simulink library "Pitch_Controller_Lib"  (R2025a)
settings: Solver=ode45  StartTime=0.0  StopTime=10.0  RelTol=1e-3  EnableMultiTasking=on
undefined symbols (not defined in the file or in its folder): Actuator_Lookup, P_VAR_Blade_Length, P_VAR_emergency_brake_pitch_angle, P_VAR_LUT_max_pitch_angle, P_VAR_park_pitch_angle, P_VAR_Rotor_nominal_rpm, PARAM_PCTRL_alpha_Igain, PARAM_PCTRL_alpha_Pgain, PARAM_PCTRL_Dgain, PARAM_PCTRL_Igain, PARAM_PCTRL_Pgain, radps2rpm, WT_Params
libraries: $bdroot x1
Description:
  | Copyright 2009-2025 The MathWorks, Inc.
settings Model: Creator=smiller  LastModifiedBy=smiller
settings SolverCC: AlgebraicLoopSolver=TrustRegion
settings DataIOCC: LimitDataPoints=on  SaveFormat=Array  SignalLoggingSaveFormat=ModelDataLogs  ReturnWorkspaceOutputs=off
settings OptimizationCC: ReuseModelBlockBuffer=off  ExpressionDepthLimit=2147483647.0  LifeSpan=inf
settings DebuggingCC: UnderspecifiedInitializationDetection=Classic  MergeDetectMultiDrivingBlocksExec=none  SolverPrmCheckMsg=warning  FcnCallInpInsideContextMsg=warning  UnconnectedInputMsg=warning  UnconnectedOutputMsg=warning  UnconnectedLineMsg=warning  AllowSymbolicDim=off  StateNameClashWarn=warning  PregeneratedLibrarySubsystemCodeDiagnostic=none  SFUnexpectedBacktrackingDiag=warning  SFNoUnconditionalDefaultTransitionDiag=warning  SFExecutionAtInitializationDiag=none  ArithmeticOperatorsInVariantConditions=warning
settings HardwareCC: ProdBitPerPointer=32.0  ProdBitPerSizeT=32.0  ProdBitPerPtrDiffT=32.0  ProdLargestAtomicFloat=None  ProdIntDivRoundTo=Undefined  ProdEndianess=Unspecified  ProdWordSize=32.0  ProdHWDeviceType=32-bit Generic
settings ModelReferenceCC: EnableRefExpFcnMdlSchedulingChecks=on  PropagateSignalLabelsOutOfModel=off
settings SFSimCC: SimUseLocalCustomCode=off  CustomCodeUndefinedFunction=UseInterfaceOnly
settings RTWCC: RTWUseLocalCustomCode=off  GPUComputeCapability=3.5  DLArmComputeVersion=19.05
settings CodeAppCC: StateflowObjectComments=on
settings GRTTargetCC: TargetLangStandard=C89/C90 (ANSI)  CombineOutputUpdateFcns=off  GRTInterface=on
settings ConfigComp: CovMetricSettings=dw  CovSaveCumulativeToWorkspaceVar=on  CovSaveSingleToWorkspaceVar=on  CovExternalEMLEnable=off  CovSFcnEnable=off

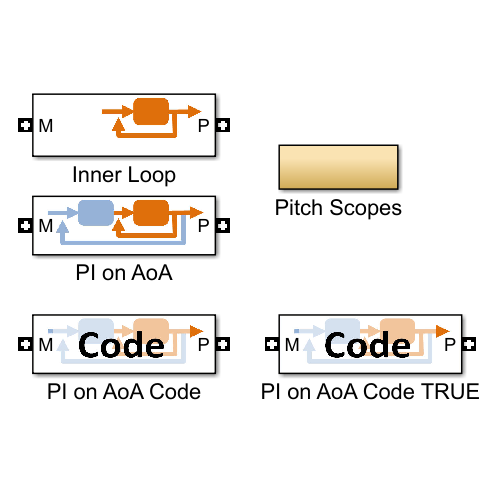
[thumbnail: Simulink's stored preview of the top-level diagram]
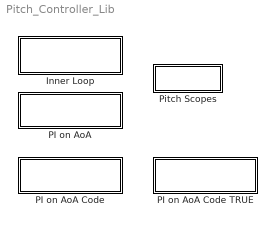
== system Pitch_Controller_Lib ==
  Inner Loop : Subsystem
      mask Display: image('Pitch_Controller_Inner_Loop_IMAGE.jpg');
  PI on AoA : Subsystem
      mask Display: image('Pitch_Controller_PI_on_AOA_IMAGE.jpg');
  PI on AoA Code : Subsystem
      mask Display: image('Pitch_Controller_PI_on_AOA_S_Function_IMAGE.jpg');
  PI on AoA Code TRUE : Subsystem
      mask Display: image('Pitch_Controller_PI_on_AOA_S_Function_IMAGE.jpg');
  Pitch Scopes : Subsystem

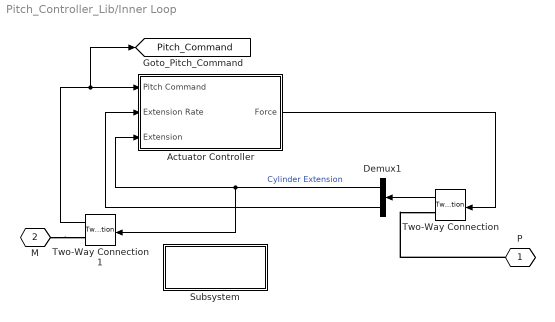
== system Pitch_Controller_Lib/Inner Loop ==
  Actuator Controller : Subsystem
  Demux1 : Demux  Outputs=2
  Subsystem : Subsystem
      mask Display: disp('Inner loop')
  Two-Way Connection : TwoWayConnection
  Two-Way Connection1 : TwoWayConnection
  P : PMIOPort  Tag=PMCPort  Side=Right
  M : PMIOPort  Tag=PMCPort  Port=2  Side=Left
  tag scope: Pitch_Command=global
  wires:
  Actuator Controller/1(Force) -> Two-Way Connection/1
  Demux1/2 -> Actuator Controller/2(Extension Rate)
  Demux1/1 -> Two-Way Connection1/1, Actuator Controller/3(Extension)  "Cylinder Extension"
  Two-Way Connection/1 -> Demux1/1
  Two-Way Connection1/1 -> [Pitch_Command], Actuator Controller/1(Pitch Command)
  connections:
  M/RConn1 -- Two-Way Connection1/RConn1
  P/RConn1 -- Two-Way Connection/RConn1

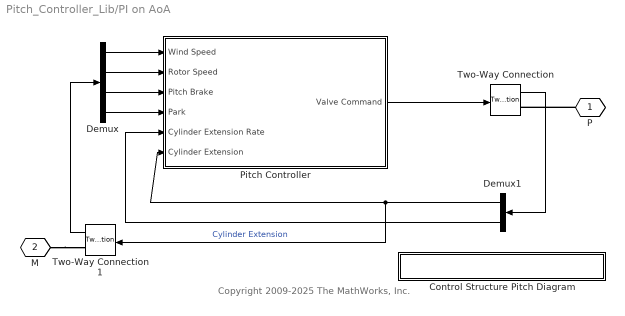
== system Pitch_Controller_Lib/PI on AoA ==
  note: Copyright 2009-2025 The MathWorks, Inc.
  Control Structure Pitch Diagram : Subsystem
      mask Display: disp('View Pitch Control Structure');
  Demux : Demux
  Demux1 : Demux  Outputs=2
  Pitch Controller : Subsystem
  Two-Way Connection : TwoWayConnection
  Two-Way Connection1 : TwoWayConnection
  P : PMIOPort  Tag=PMCPort  Side=Right
  M : PMIOPort  Tag=PMCPort  Port=2  Side=Left
  wires:
  Pitch Controller/1(Valve Command) -> Two-Way Connection/1
  Two-Way Connection/1 -> Demux1/1
  Demux1/2 -> Pitch Controller/5(Cylinder Extension Rate)
  Demux1/1 -> Two-Way Connection1/1, Pitch Controller/6(Cylinder Extension)  "Cylinder Extension"
  Two-Way Connection1/1 -> Demux/1
  Demux/1 -> Pitch Controller/1(Wind Speed)
  Demux/2 -> Pitch Controller/2(Rotor Speed)
  Demux/3 -> Pitch Controller/3(Pitch Brake)
  Demux/4 -> Pitch Controller/4(Park)
  connections:
  P/RConn1 -- Two-Way Connection/RConn1
  M/RConn1 -- Two-Way Connection1/RConn1

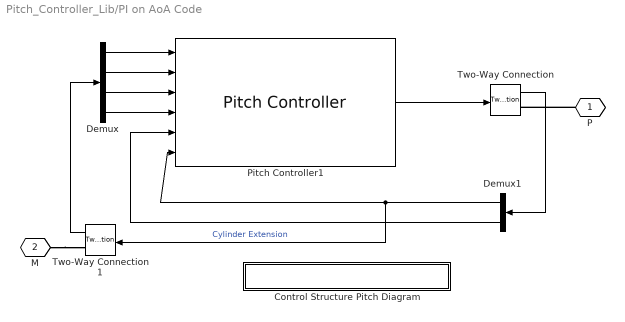
== system Pitch_Controller_Lib/PI on AoA Code ==
  Control Structure Pitch Diagram : Subsystem
      mask Display: disp('View Pitch Control Structure');
  Demux : Demux
  Demux1 : Demux  Outputs=2
  Pitch Controller1 : $bdroot/PI on AoA/Pitch Controller  SystemSampleTime=-1  VariantActivationTime=update diagram  EmptyChoice=off  PassThrough=off  PassThroughVariantControl=(default)  EmptyChoiceVariantControl=(default)  AllowFlexibleInterface=on  Latency=0  AutoFrameSizeCalculation=off
  Two-Way Connection : TwoWayConnection
  Two-Way Connection1 : TwoWayConnection
  P : PMIOPort  Tag=PMCPort  Side=Right
  M : PMIOPort  Tag=PMCPort  Port=2  Side=Left
  wires:
  Demux/4 -> Pitch Controller1/4
  Demux/3 -> Pitch Controller1/3
  Demux/2 -> Pitch Controller1/2
  Demux/1 -> Pitch Controller1/1
  Two-Way Connection1/1 -> Demux/1
  Demux1/1 -> Pitch Controller1/6, Two-Way Connection1/1  "Cylinder Extension"
  Demux1/2 -> Pitch Controller1/5
  Two-Way Connection/1 -> Demux1/1
  Pitch Controller1/1 -> Two-Way Connection/1
  connections:
  M/RConn1 -- Two-Way Connection1/RConn1
  P/RConn1 -- Two-Way Connection/RConn1

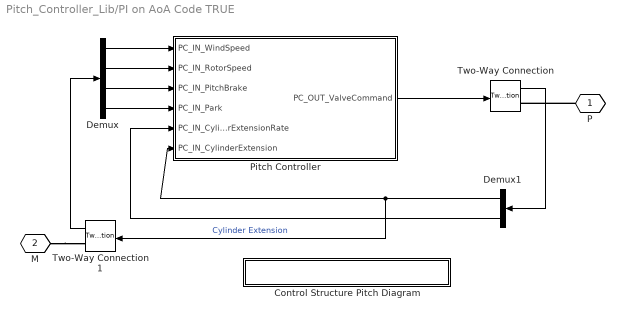
== system Pitch_Controller_Lib/PI on AoA Code TRUE ==
  Control Structure Pitch Diagram : Subsystem
      mask Display: disp('View Pitch Control Structure');
  Demux : Demux
  Demux1 : Demux  Outputs=2
  Pitch Controller : Subsystem
  Two-Way Connection : TwoWayConnection
  Two-Way Connection1 : TwoWayConnection
  P : PMIOPort  Tag=PMCPort  Side=Right
  M : PMIOPort  Tag=PMCPort  Port=2  Side=Left
  wires:
  Pitch Controller/1(PC_OUT_ValveCommand) -> Two-Way Connection/1
  Two-Way Connection/1 -> Demux1/1
  Demux1/2 -> Pitch Controller/5(PC_IN_CylinderExtensionRate)
  Demux1/1 -> Pitch Controller/6(PC_IN_CylinderExtension), Two-Way Connection1/1  "Cylinder Extension"
  Two-Way Connection1/1 -> Demux/1
  Demux/1 -> Pitch Controller/1(PC_IN_WindSpeed)
  Demux/2 -> Pitch Controller/2(PC_IN_RotorSpeed)
  Demux/3 -> Pitch Controller/3(PC_IN_PitchBrake)
  Demux/4 -> Pitch Controller/4(PC_IN_Park)
  connections:
  P/RConn1 -- Two-Way Connection/RConn1
  M/RConn1 -- Two-Way Connection1/RConn1

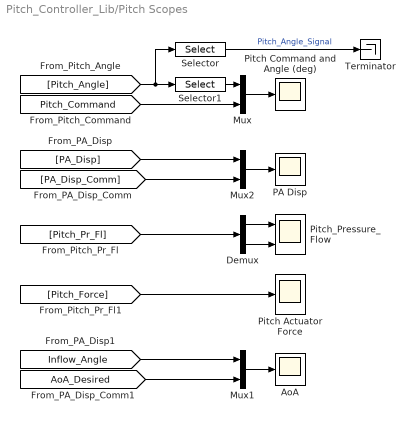
== system Pitch_Controller_Lib/Pitch Scopes ==
  AoA : Scope
      settings: TimeSpan=10  ActiveDisplayYMinimum=-1.6  ActiveDisplayYMaximum=-0.9  DataLoggingVariableName=ScopeData2
  Demux : Demux  Outputs=[2 1]
  Mux : Mux  Inputs=2
  Mux1 : Mux  Inputs=2
  Mux2 : Mux  Inputs=2
  PA Disp : Scope
      settings: TimeSpan=10  ActiveDisplayYMinimum=-1.6  ActiveDisplayYMaximum=-0.9
  Pitch Actuator Force : Scope
      settings: TimeSpan=80  ActiveDisplayYMinimum=-78125  ActiveDisplayYMaximum=84375  DataLoggingVariableName=Pitch_Actuator_Force_DATA
  Pitch Command and Angle (deg) : Scope
      settings: TimeSpan=80  ActiveDisplayYMinimum=-20  ActiveDisplayYMaximum=80  DataLoggingVariableName=Blade_Pitch_DATA
  Pitch_Pressure_Flow : Scope  NumInputPorts=2
      settings: ActiveDisplayYMinimum=-5  ActiveDisplayYMaximum=20  DataLoggingVariableName=ScopeData3
  Selector : Selector  InputPortWidth=3  IndexOptions=Index vector (dialog)  Indices=[1 ]  OutputSizes=1
  Selector1 : Selector  InputPortWidth=3  IndexOptions=Index vector (dialog)  Indices=[1 ]  OutputSizes=1
  Terminator : Terminator
  wires:
  Selector1/1 -> Mux/1
  [Inflow_Angle] -> Mux1/1
  Mux1/1 -> AoA/1
  [AoA_Desired] -> Mux1/2
  [Pitch_Angle] -> Selector1/1, Selector/1
  [Pitch_Command] -> Mux/2
  Mux/1 -> Pitch Command and Angle (deg)/1
  [PA_Disp] -> Mux2/1
  Mux2/1 -> PA Disp/1
  [PA_Disp_Comm] -> Mux2/2
  [Pitch_Pr_Fl] -> Demux/1
  Demux/1 -> Pitch_Pressure_Flow/1
  Demux/2 -> Pitch_Pressure_Flow/2
  Selector/1 -> Terminator/1  "Pitch_Angle_Signal"
  [Pitch_Force] -> Pitch Actuator Force/1

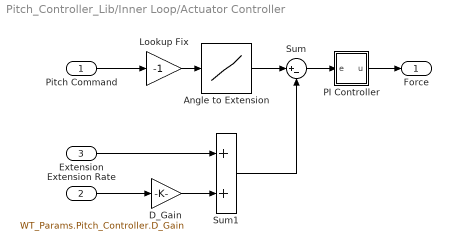
== system Pitch_Controller_Lib/Inner Loop/Actuator Controller ==
  Pitch Command : Inport
  Extension Rate : Inport  Port=2
  Extension : Inport  Port=3
  Angle to Extension : Lookup  InputValues=-Actuator_Lookup.angle  Table=Actuator_Lookup.extension  SaturateOnIntegerOverflow=off
  D_Gain : Gain  Gain=WT_Params.Pitch_Controller.D_Gain
  Lookup Fix : Gain  Gain=-1
  PI Controller : Subsystem
      mask Display: disp('PI')
  Sum : Sum  Inputs=|+-
  Sum1 : Sum
  Force : Outport  VectorParamsAs1DForOutWhenUnconnected=off
  wires:
  Extension Rate/1 -> D_Gain/1
  PI Controller/1(u) -> Force/1
  Extension/1 -> Sum1/1
  Pitch Command/1 -> Lookup Fix/1
  Sum1/1 -> Sum/2
  D_Gain/1 -> Sum1/2
  Lookup Fix/1 -> Angle to Extension/1
  Angle to Extension/1 -> Sum/1
  Sum/1 -> PI Controller/1(e)

== system Pitch_Controller_Lib/Inner Loop/Subsystem ==

== system Pitch_Controller_Lib/PI on AoA/Control Structure Pitch Diagram ==
  Subsystem : Subsystem
      mask Display: image(imread('Control_Structure_Pitch_IMAGE.jpg'));

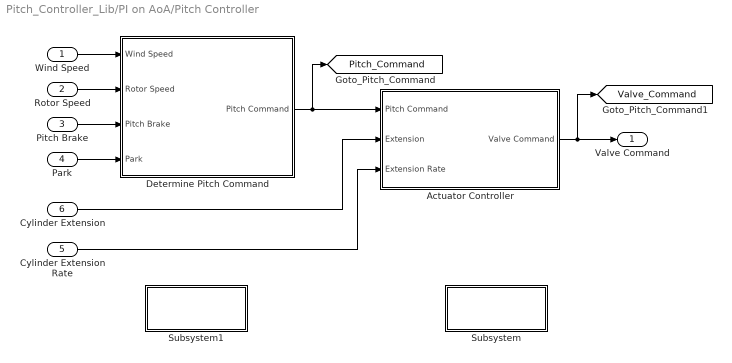
== system Pitch_Controller_Lib/PI on AoA/Pitch Controller ==
  Wind Speed : Inport
  Rotor Speed : Inport  Port=2
  Pitch Brake : Inport  Port=3
  Park : Inport  Port=4
  Cylinder Extension Rate : Inport  Port=5
  Cylinder Extension : Inport  Port=6
  Actuator Controller : Subsystem
  Determine Pitch Command : Subsystem
  Subsystem : Subsystem
      mask Display: disp('Inner loop')
  Subsystem1 : Subsystem
      mask Display: disp('Outer loop')
  Valve Command : Outport  VectorParamsAs1DForOutWhenUnconnected=off
  tag scope: Pitch_Command=global, Valve_Command=global
  wires:
  Determine Pitch Command/1(Pitch Command) -> [Pitch_Command], Actuator Controller/1(Pitch Command)
  Cylinder Extension/1 -> Actuator Controller/2(Extension)
  Wind Speed/1 -> Determine Pitch Command/1(Wind Speed)
  Rotor Speed/1 -> Determine Pitch Command/2(Rotor Speed)
  Actuator Controller/1(Valve Command) -> Valve Command/1, [Valve_Command]
  Pitch Brake/1 -> Determine Pitch Command/3(Pitch Brake)
  Park/1 -> Determine Pitch Command/4(Park)
  Cylinder Extension Rate/1 -> Actuator Controller/3(Extension Rate)

== system Pitch_Controller_Lib/PI on AoA Code/Control Structure Pitch Diagram ==
  Subsystem : Subsystem
      mask Display: image(imread('Control_Structure_Pitch_IMAGE.jpg'));

== system Pitch_Controller_Lib/PI on AoA Code TRUE/Control Structure Pitch Diagram ==
  Subsystem : Subsystem
      mask Display: image(imread('Control_Structure_Pitch_IMAGE.jpg'));

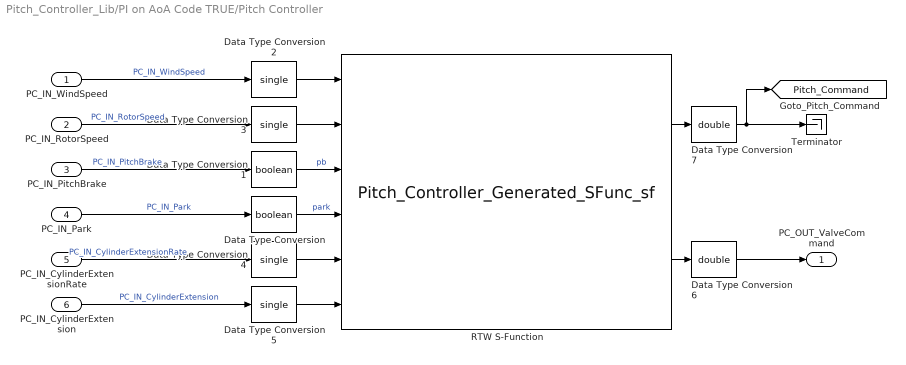
== system Pitch_Controller_Lib/PI on AoA Code TRUE/Pitch Controller ==
  PC_IN_WindSpeed : Inport  OutDataTypeStr=double
  PC_IN_RotorSpeed : Inport  Port=2  OutDataTypeStr=double
  PC_IN_PitchBrake : Inport  Port=3  OutDataTypeStr=double
  PC_IN_Park : Inport  Port=4  OutDataTypeStr=double
  PC_IN_CylinderExtensionRate : Inport  Port=5  OutDataTypeStr=double  PortDimensions=3
  PC_IN_CylinderExtension : Inport  Port=6  OutDataTypeStr=double  PortDimensions=3
  Data Type Conversion : DataTypeConversion  OutDataTypeStr=boolean  SaturateOnIntegerOverflow=off  RndMeth=Floor
  Data Type Conversion1 : DataTypeConversion  OutDataTypeStr=boolean  SaturateOnIntegerOverflow=off  RndMeth=Floor
  Data Type Conversion{2..5} (4 alike) : DataTypeConversion  OutDataTypeStr=single  SaturateOnIntegerOverflow=off  RndMeth=Floor
  Data Type Conversion6 : DataTypeConversion  OutDataTypeStr=double  SaturateOnIntegerOverflow=off  RndMeth=Floor
  Data Type Conversion7 : DataTypeConversion  OutDataTypeStr=double  SaturateOnIntegerOverflow=off  RndMeth=Floor
  RTW S-Function : S-Function  FunctionName=Pitch_Controller_Generated_SFunc_sf  Parameters=sfcnParam1, sfcnParam2, sfcnParam3, sfcnParam4, sfcnParam5, sfcnParam6, sfcnParam7, sfcnParam8, sfcnParam9, sfcnParam10  SFunctionModules=""  SFunctionDeploymentMode=off  EnableBusSupport=off  mask{rtw_sf_name=Pitch_Controller_Generated_SFunc_sf, showVar=off, sfcnParam1=PARAM_PCTRL_Dgain, sfcnParam2=PARAM_PCTRL_Igain, sfcnParam3=PARAM_PCTRL_Pgain, sfcnParam4=PARAM_PCTRL_alpha_Igain, sfcnParam5=PARAM_PCTRL_alpha_Pgain, sfcnParam6=P_VAR_Blade_Length, sfcnParam7=P_VAR_LUT_max_pitch_angle, sfcnParam8=P_VAR_Rotor_nominal_rpm, sfcnParam9=P_VAR_emergency_brake_pitch_angle, sfcnParam10=P_VAR_park_pitch_angle}
      mask prompts: rtw_sf_name "Generated S-function name (model_sf):"; showVar "Show module list"; sfcnParam1 "PARAM_PCTRL_Dgain:"; sfcnParam2 "PARAM_PCTRL_Igain:"; sfcnParam3 "PARAM_PCTRL_Pgain:"; sfcnParam4 "PARAM_PCTRL_alpha_Igain:"; sfcnParam5 "PARAM_PCTRL_alpha_Pgain:"; sfcnParam6 "P_VAR_Blade_Length:"; sfcnParam7 "P_VAR_LUT_max_pitch_angle:"; sfcnParam8 "P_VAR_Rotor_nominal_rpm:"; sfcnParam9 "P_VAR_emergency_brake_pitch_angle:"; sfcnParam10 "P_VAR_park_pitch_angle:"
      mask help: Real-Time Workshop generated S-function.
      mask init:
      | displist = '';
      | if ~strcmp(get_param(gcb, 'FunctionName'), rtw_sf_name);
      |   set_param(gcb, 'FunctionName', rtw_sf_name);
      | end
      | % Check if we are generating RTW code
      | rtw_mode = false;
      | if strcmpi(get_param(bdroot(gcb),'SimulationStatus'),'Initializing')
      | 	rtw_mode = strcmpi(get_param(bdroot(gcb),'BuildingRTWCode'),'on') && ...
      | 		~strcmpi(get_param(bdroot(gcb),'TargetStyle'),'SimulationTarget');
      | end
      | if showVar || rtw_mode
      | 	if exist('rtwsfunc') == 2 | exist('rtwsfunc') == 6
      | 		tmplist = rtwsfunc(rtw_sf_name,gcb);
      | 		tmplist = ['\nList of Modules:\n', tmplist];
      | 	elseif showVar
      | 		tmplist = '\nList of Modules:\nRTW not licensed\n';
      |  	end
      | end
      | if showVar
      |   displist = tmplist;
      | end
      settings: CopyFcn=|
      | if ~strcmp(get_param(gcb,'Linkstatus'),'none') && ...
      | ~strcmp(get_param(gcb,'Linkstatus'),'implicit')
      |   set_param(gcb,'LinkStatus','none');
      | end
      mask Help: eval('feval(''rtwprivate'',''rtwhelpview'',''rtw_sfcn_block'')');
      mask Display:
      | port_label('input',1,'PC_IN_WindSpeed');
      | port_label('input',2,'PC_IN_RotorSpeed');
      | port_label('input',3,'PC_IN_PitchBrake');
      | port_label('input',4,'PC_IN_Park');
      | port_label('input',5,'PC_IN_CylinderExtensionRate');
      | port_label('input',6,'PC_IN_CylinderExtension');
      | port_label('output',1,'PC_LOG_PitchCommand');
      | port_label('output',2,'PC_OUT_ValveCommand');
  Terminator : Terminator
  PC_OUT_ValveCommand : Outport  OutDataTypeStr=double  VectorParamsAs1DForOutWhenUnconnected=off
  tag scope: Pitch_Command=global
  wires:
  Data Type Conversion7/1 -> [Pitch_Command], Terminator/1
  RTW S-Function/1 -> Data Type Conversion7/1
  RTW S-Function/2 -> Data Type Conversion6/1
  Data Type Conversion6/1 -> PC_OUT_ValveCommand/1
  Data Type Conversion5/1 -> RTW S-Function/6
  Data Type Conversion4/1 -> RTW S-Function/5
  Data Type Conversion3/1 -> RTW S-Function/2
  Data Type Conversion2/1 -> RTW S-Function/1
  Data Type Conversion1/1 -> RTW S-Function/3  "pb"
  Data Type Conversion/1 -> RTW S-Function/4  "park"
  PC_IN_CylinderExtension/1 -> Data Type Conversion5/1  "PC_IN_CylinderExtension"
  PC_IN_CylinderExtensionRate/1 -> Data Type Conversion4/1  "PC_IN_CylinderExtensionRate"
  PC_IN_Park/1 -> Data Type Conversion/1  "PC_IN_Park"
  PC_IN_PitchBrake/1 -> Data Type Conversion1/1  "PC_IN_PitchBrake"
  PC_IN_RotorSpeed/1 -> Data Type Conversion3/1  "PC_IN_RotorSpeed"
  PC_IN_WindSpeed/1 -> Data Type Conversion2/1  "PC_IN_WindSpeed"

== system Pitch_Controller_Lib/Inner Loop/Actuator Controller/PI Controller ==
  e : Inport
  Integral Gain : Gain  Gain=WT_Params.Pitch_Controller.I_Gain  SaturateOnIntegerOverflow=on  OutDataTypeStr=Inherit: Same as input  ParamDataTypeStr=Inherit: Same as input
  Integrator : Integrator
  Proportional Gain : Gain  Gain=WT_Params.Pitch_Controller.P_Gain  SaturateOnIntegerOverflow=on  OutDataTypeStr=Inherit: Same as input  ParamDataTypeStr=Inherit: Same as input
  Sum : Sum  Inputs=++|  InputSameDT=on  SaturateOnIntegerOverflow=on  OutDataTypeStr=Inherit: Same as first input
  u : Outport  InitialOutput=0  VectorParamsAs1DForOutWhenUnconnected=off
  wires:
  Sum/1 -> u/1
  e/1 -> Integral Gain/1, Proportional Gain/1
  Integrator/1 -> Sum/2
  Proportional Gain/1 -> Sum/1
  Integral Gain/1 -> Integrator/1

== system Pitch_Controller_Lib/PI on AoA/Control Structure Pitch Diagram/Subsystem ==

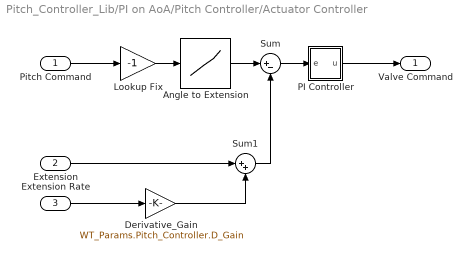
== system Pitch_Controller_Lib/PI on AoA/Pitch Controller/Actuator Controller ==
  Pitch Command : Inport
  Extension : Inport  Port=2
  Extension Rate : Inport  Port=3
  Angle to Extension : Lookup  InputValues=-Actuator_Lookup.angle  Table=Actuator_Lookup.extension  LookUpMeth=Interpolation-Use End Values  SaturateOnIntegerOverflow=off
  Derivative_Gain : Gain  Gain=WT_Params.Pitch_Controller.D_Gain
  Lookup Fix : Gain  Gain=-1
  PI Controller : Subsystem
      mask Display: disp('PI')
  Sum : Sum  Inputs=|+-
  Sum1 : Sum  Inputs=|++
  Valve Command : Outport  VectorParamsAs1DForOutWhenUnconnected=off
  wires:
  Sum1/1 -> Sum/2
  Derivative_Gain/1 -> Sum1/2
  Lookup Fix/1 -> Angle to Extension/1
  Angle to Extension/1 -> Sum/1
  Sum/1 -> PI Controller/1(e)
  Pitch Command/1 -> Lookup Fix/1
  PI Controller/1(u) -> Valve Command/1
  Extension/1 -> Sum1/1
  Extension Rate/1 -> Derivative_Gain/1

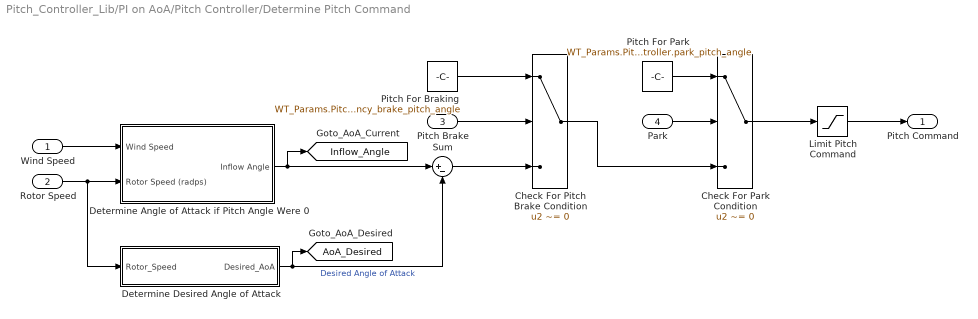
== system Pitch_Controller_Lib/PI on AoA/Pitch Controller/Determine Pitch Command ==
  Wind Speed : Inport
  Rotor Speed : Inport  Port=2
  Pitch Brake : Inport  Port=3
  Park : Inport  Port=4
  Check For Park Condition : Switch  Criteria=u2 ~= 0  SaturateOnIntegerOverflow=off  InputSameDT=off
  Check For Pitch Brake Condition : Switch  Criteria=u2 ~= 0  SaturateOnIntegerOverflow=off  InputSameDT=off
  Determine Angle of Attack if Pitch Angle Were 0 : Subsystem
  Determine Desired Angle of Attack : Subsystem
  Limit Pitch Command : Saturate  UpperLimit=max(Actuator_Lookup.angle)  LowerLimit=WT_Params.Pitch_Controller.emergency_brake_pitch_angle
  Pitch For Braking : Constant  Value=WT_Params.Pitch_Controller.emergency_brake_pitch_angle
  Pitch For Park : Constant  Value=WT_Params.Pitch_Controller.park_pitch_angle
  Sum : Sum  Inputs=|+-
  Pitch Command : Outport  VectorParamsAs1DForOutWhenUnconnected=off
  tag scope: AoA_Desired=global, Inflow_Angle=global
  wires:
  Limit Pitch Command/1 -> Pitch Command/1
  Wind Speed/1 -> Determine Angle of Attack if Pitch Angle Were 0/1(Wind Speed)
  Rotor Speed/1 -> Determine Desired Angle of Attack/1(Rotor_Speed), Determine Angle of Attack if Pitch Angle Were 0/2(Rotor Speed (radps))
  Determine Angle of Attack if Pitch Angle Were 0/1(Inflow Angle) -> Sum/1, [Inflow_Angle]
  Determine Desired Angle of Attack/1(Desired_AoA) -> Sum/2, [AoA_Desired]  "Desired Angle of Attack"
  Sum/1 -> Check For Pitch Brake Condition/3
  Pitch Brake/1 -> Check For Pitch Brake Condition/2
  Pitch For Braking/1 -> Check For Pitch Brake Condition/1
  Park/1 -> Check For Park Condition/2
  Pitch For Park/1 -> Check For Park Condition/1
  Check For Pitch Brake Condition/1 -> Check For Park Condition/3
  Check For Park Condition/1 -> Limit Pitch Command/1

== system Pitch_Controller_Lib/PI on AoA/Pitch Controller/Subsystem ==

== system Pitch_Controller_Lib/PI on AoA/Pitch Controller/Subsystem1 ==

== system Pitch_Controller_Lib/PI on AoA Code/Control Structure Pitch Diagram/Subsystem ==

== system Pitch_Controller_Lib/PI on AoA Code TRUE/Control Structure Pitch Diagram/Subsystem ==

== system Pitch_Controller_Lib/PI on AoA/Pitch Controller/Actuator Controller/PI Controller ==
  e : Inport
  Integral Gain : Gain  Gain=WT_Params.Pitch_Controller.I_Gain  SaturateOnIntegerOverflow=on  OutDataTypeStr=Inherit: Same as input  ParamDataTypeStr=Inherit: Same as input
  Integrator : Integrator
  Proportional Gain : Gain  Gain=WT_Params.Pitch_Controller.P_Gain  SaturateOnIntegerOverflow=on  OutDataTypeStr=Inherit: Same as input  ParamDataTypeStr=Inherit: Same as input
  Sum : Sum  Inputs=++|  InputSameDT=on  SaturateOnIntegerOverflow=on  OutDataTypeStr=Inherit: Same as first input
  u : Outport  InitialOutput=0  VectorParamsAs1DForOutWhenUnconnected=off
  wires:
  Sum/1 -> u/1
  e/1 -> Integral Gain/1, Proportional Gain/1
  Integrator/1 -> Sum/2
  Proportional Gain/1 -> Sum/1
  Integral Gain/1 -> Integrator/1

== system Pitch_Controller_Lib/PI on AoA/Pitch Controller/Determine Pitch Command/Determine Angle of Attack if Pitch Angle Were 0 ==
  Wind Speed : Inport
  Rotor Speed (radps) : Inport  Port=2
  Trigonometric Function : Trigonometry  Operator=atan2
  rad2deg : Gain  Gain=180/pi
  radps2mps : Gain  Gain=WT_Params.Blade.length
  Inflow Angle : Outport  VectorParamsAs1DForOutWhenUnconnected=off
  tag scope: Max_Chord_Speed=global
  wires:
  rad2deg/1 -> Inflow Angle/1
  Rotor Speed (radps)/1 -> radps2mps/1
  Wind Speed/1 -> Trigonometric Function/1
  Trigonometric Function/1 -> rad2deg/1
  radps2mps/1 -> Trigonometric Function/2, [Max_Chord_Speed]

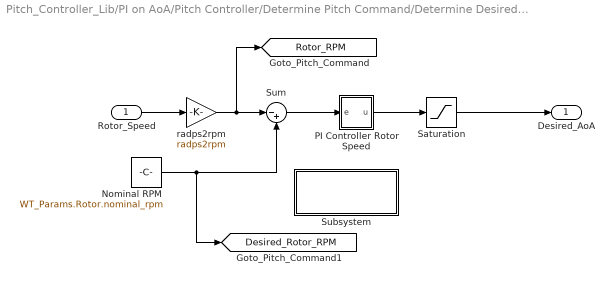
== system Pitch_Controller_Lib/PI on AoA/Pitch Controller/Determine Pitch Command/Determine Desired Angle of Attack ==
  Rotor_Speed : Inport
  Nominal RPM : Constant  Value=WT_Params.Rotor.nominal_rpm
  PI Controller Rotor Speed : Subsystem
      mask Display:
      | plot([0 1],[0 0]);
      | plot([1 2],[0 1]);
      | plot([2 3],[1 1]);
      | disp('P I');
  Saturation : Saturate  UpperLimit=WT_Params.Pitch_Controller.Angle_Of_Attack.max_angle  LowerLimit=-inf
  Subsystem : Subsystem
      mask Display: disp('Outer loop')
  Sum : Sum  Inputs=|-+
  radps2rpm : Gain  Gain=radps2rpm
  Desired_AoA : Outport  VectorParamsAs1DForOutWhenUnconnected=off
  tag scope: Desired_Rotor_RPM=global, Rotor_RPM=global
  wires:
  Saturation/1 -> Desired_AoA/1
  Rotor_Speed/1 -> radps2rpm/1
  PI Controller Rotor Speed/1(u) -> Saturation/1
  radps2rpm/1 -> [Rotor_RPM], Sum/1
  Nominal RPM/1 -> [Desired_Rotor_RPM], Sum/2
  Sum/1 -> PI Controller Rotor Speed/1(e)

== system Pitch_Controller_Lib/PI on AoA/Pitch Controller/Determine Pitch Command/Determine Desired Angle of Attack/PI Controller Rotor Speed ==
  e : Inport
  Integral Gain : Gain  Gain=WT_Params.Pitch_Controller.Angle_Of_Attack.I_Gain  SaturateOnIntegerOverflow=on  OutDataTypeStr=Inherit: Same as input  ParamDataTypeStr=Inherit: Same as input
  Integrator : Integrator  LimitOutput=on  UpperSaturationLimit=WT_Params.Pitch_Controller.Angle_Of_Attack.max_angle  LowerSaturationLimit=-WT_Params.Pitch_Controller.Angle_Of_Attack.max_angle
  Proportional Gain : Gain  Gain=WT_Params.Pitch_Controller.Angle_Of_Attack.P_Gain  SaturateOnIntegerOverflow=on  OutDataTypeStr=Inherit: Same as input  ParamDataTypeStr=Inherit: Same as input
  Sum : Sum  Inputs=++|  InputSameDT=on  SaturateOnIntegerOverflow=on  OutDataTypeStr=Inherit: Same as first input
  u : Outport  InitialOutput=0  VectorParamsAs1DForOutWhenUnconnected=off
  wires:
  e/1 -> Integral Gain/1, Proportional Gain/1
  Integrator/1 -> Sum/2
  Proportional Gain/1 -> Sum/1
  Integral Gain/1 -> Integrator/1
  Sum/1 -> u/1

== system Pitch_Controller_Lib/PI on AoA/Pitch Controller/Determine Pitch Command/Determine Desired Angle of Attack/Subsystem ==
